simulink model "closed_loop_discrete"  (R2024b)
settings: Solver=FixedStepDiscrete  StartTime=0.0  StopTime=0.6  FixedStep=5e-05  RelTol=1e-3
settings Model: Creator=m1516  LastModifiedBy=m1516
settings DataIOCC: SignalLogging=off

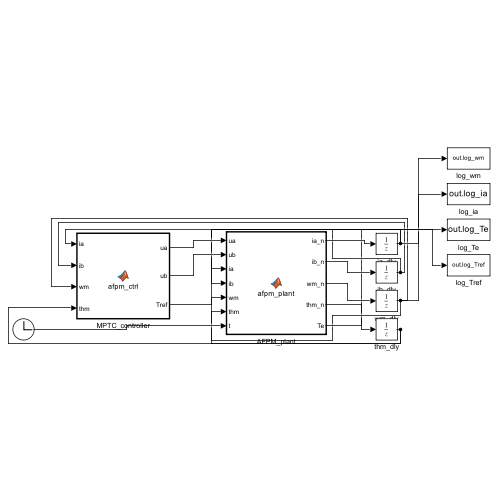
[thumbnail: Simulink's stored preview of the top-level diagram]
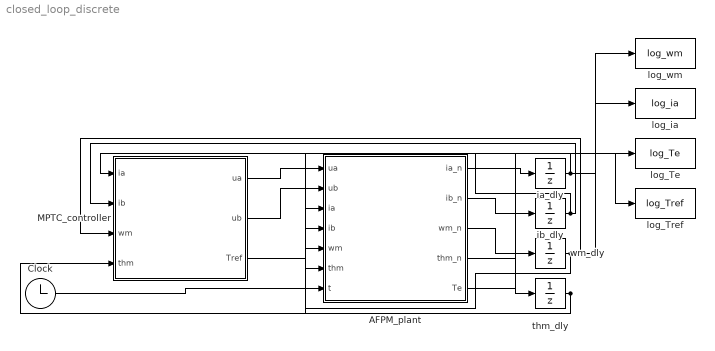
== system closed_loop_discrete ==
  AFPM_plant : MATLAB Function  TreatAsAtomicUnit=on
  Clock : Clock
  MPTC_controller : MATLAB Function  TreatAsAtomicUnit=on
  ia_dly : UnitDelay  SampleTime=5e-05  HasFrameUpgradeWarning=on
  ib_dly : UnitDelay  SampleTime=5e-05  HasFrameUpgradeWarning=on
  log_Te : ToWorkspace  VariableName=log_Te  SaveFormat=Structure With Time  SampleTime=5e-05
  log_Tref : ToWorkspace  VariableName=log_Tref  SaveFormat=Structure With Time  SampleTime=5e-05
  log_ia : ToWorkspace  VariableName=log_ia  SaveFormat=Structure With Time  SampleTime=5e-05
  log_wm : ToWorkspace  VariableName=log_wm  SaveFormat=Structure With Time  SampleTime=5e-05
  thm_dly : UnitDelay  SampleTime=5e-05  HasFrameUpgradeWarning=on
  wm_dly : UnitDelay  SampleTime=5e-05  HasFrameUpgradeWarning=on
  wires:
  Clock/1 -> AFPM_plant/7(t)
  MPTC_controller/1(ua) -> AFPM_plant/1(ua)
  MPTC_controller/2(ub) -> AFPM_plant/2(ub)
  ia_dly/1 -> MPTC_controller/1(ia), AFPM_plant/3(ia), log_ia/1
  ib_dly/1 -> MPTC_controller/2(ib), AFPM_plant/4(ib)
  wm_dly/1 -> MPTC_controller/3(wm), AFPM_plant/5(wm), log_wm/1
  thm_dly/1 -> MPTC_controller/4(thm), AFPM_plant/6(thm)
  AFPM_plant/1(ia_n) -> ia_dly/1
  AFPM_plant/2(ib_n) -> ib_dly/1
  AFPM_plant/3(wm_n) -> wm_dly/1
  AFPM_plant/4(thm_n) -> thm_dly/1
  AFPM_plant/5(Te) -> log_Te/1
  MPTC_controller/3(Tref) -> log_Tref/1

== matlab function closed_loop_discrete/AFPM_plant ==
  settings: updateMethod=DISCRETE  sampleTime=5e-05
  data: ua input; ia_n output; ub input; ia input; ib input; wm input; thm input; t input; ib_n output; wm_n output; thm_n output; Te output
function [ia_n,ib_n,wm_n,thm_n,Te] = afpm_plant(ua,ub,ia,ib,wm,thm,t)
%#codegen
Rs=0.2; L=0.0085; psi=0.175; p=4; J=0.003; F=0.008; Ts=5e-05; Ns=20;
Tload=8; tstep=0.3;
h = Ts/Ns;
% 转矩按块输入（步初）状态计算，使 Te 与同索引的 ia/wm 处于同一时刻口径。
Te = 1.5*p*psi*(-ia*sin(p*thm) + ib*cos(p*thm));
for k = 1:Ns
    tk = t + (k-1)*h;
    tl = double(tk + 0.5*h >= tstep)*Tload;
    [k1a,k1b,k1w,k1t] = f(ia,ib,wm,thm,ua,ub,tl,Rs,L,psi,p,J,F);
    [k2a,k2b,k2w,k2t] = f(ia+.5*h*k1a,ib+.5*h*k1b,wm+.5*h*k1w,thm+.5*h*k1t,ua,ub,tl,Rs,L,psi,p,J,F);
    [k3a,k3b,k3w,k3t] = f(ia+.5*h*k2a,ib+.5*h*k2b,wm+.5*h*k2w,thm+.5*h*k2t,ua,ub,tl,Rs,L,psi,p,J,F);
    [k4a,k4b,k4w,k4t] = f(ia+h*k3a,ib+h*k3b,wm+h*k3w,thm+h*k3t,ua,ub,tl,Rs,L,psi,p,J,F);
    ia = ia + h/6*(k1a+2*k2a+2*k3a+k4a);
    ib = ib + h/6*(k1b+2*k2b+2*k3b+k4b);
    wm = wm + h/6*(k1w+2*k2w+2*k3w+k4w);
    thm = thm + h/6*(k1t+2*k2t+2*k3t+k4t);
end
ia_n = ia; ib_n = ib; wm_n = wm; thm_n = thm;
end
function [da,db,dw,dt] = f(ia,ib,wm,thm,ua,ub,tl,Rs,L,psi,p,J,F)
te = 1.5*p*psi*(-ia*sin(p*thm) + ib*cos(p*thm));
da = (ua - Rs*ia + psi*p*wm*sin(p*thm))/L;
db = (ub - Rs*ib - psi*p*wm*cos(p*thm))/L;
dw = (te - tl - F*wm)/J;
dt = wm;
end

== matlab function closed_loop_discrete/MPTC_controller ==
  settings: updateMethod=DISCRETE  sampleTime=5e-05
  data: ia input; ua output; ib input; wm input; thm input; ub output; Tref output
function [ua,ub,Tref] = afpm_ctrl(ia,ib,wm,thm)
%#codegen
persistent pend iw cost
if isempty(pend)
    pend = 7; iw = 0; cost = zeros(1,8);
end
Rs=0.2; L=0.0085; psi=0.175; p=4; Ts=5e-05; Udc=250;
wref=31.4159265359; Kp=2; Ki=8; Tr=11.9; lf=1; lsw=0.02;
V = [166.666666667 0;83.3333333333 144.337567297;-83.3333333333 144.337567297;-166.666666667 0;-83.3333333333 -144.337567297;83.3333333333 -144.337567297;0 0;0 0];
S = [1 0 0;1 1 0;0 1 0;0 1 1;0 0 1;1 0 1;0 0 0;1 1 1] > 0.5;
Tcap = 1.5*Tr;
ew = wref - wm; raw = Kp*ew + iw;
Tref = min(max(raw,-Tcap),Tcap);
if abs(raw) <= Tcap || raw*ew < 0
    iw = iw + Ki*ew*Ts;
end
ua = V(pend,1); ub = V(pend,2);
theta = p*thm; we = p*wm;
xa = ia; xb = ib;
% 一拍延时补偿：先按本拍施加的矢量前推一拍
xa = xa + Ts*(ua - Rs*xa + psi*we*sin(theta))/L;
xb = xb + Ts*(ub - Rs*xb - psi*we*cos(theta))/L;
theta = theta + Ts*we;
for k = 1:8
    a2 = xa + Ts*(V(k,1) - Rs*xa + psi*we*sin(theta))/L;
    b2 = xb + Ts*(V(k,2) - Rs*xb - psi*we*cos(theta))/L;
    t2 = theta + Ts*we;
    pa = L*a2 + psi*cos(t2); pb = L*b2 + psi*sin(t2);
    Tp = 1.5*p*psi*(-a2*sin(t2) + b2*cos(t2));
    flips = sum(S(k,:) ~= S(pend,:));
    cost(k) = abs(Tref - Tp)/Tr + lf*abs(hypot(pa,pb) - psi)/psi + lsw*flips;
end
[~, cv] = min(cost);
pend = cv;
end
